simulink model "bolid_sim_2"  (R2026b)
settings: Solver=ode23t  StopTime=180
model workspace (MAT data in the model file):
  sample_time = 0.001
libraries: fl_lib x19, nesl_utility x14, ee_lib x6, slpidlib x2, simulink x1, sdl_lib x1
settings Model: Creator=LH213  LastModifiedBy=stycz
settings RTWCC: GPUComputeCapability=5.0
settings SimscapeCC: SimscapeUseEnergyAccounting=off

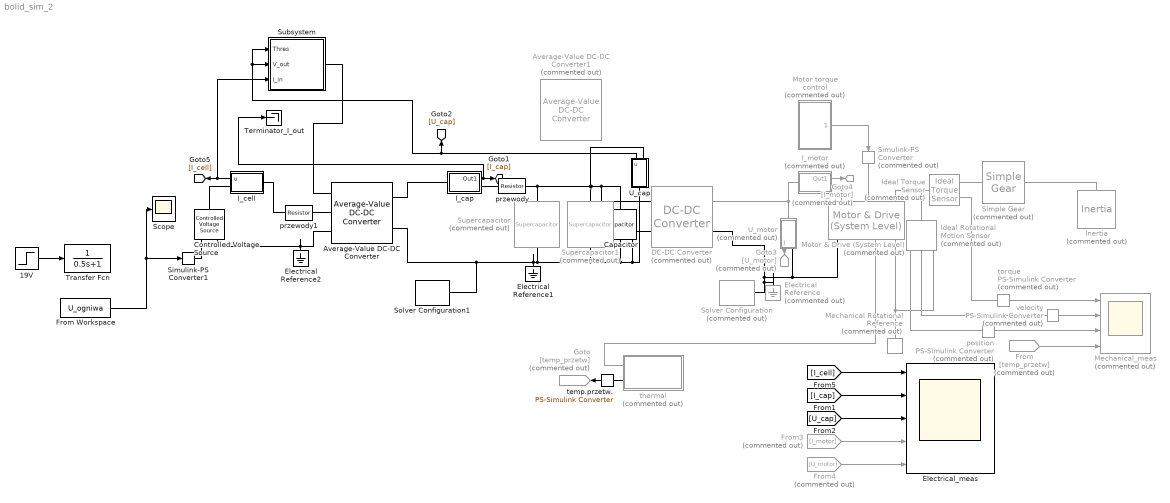
== system bolid_sim_2 ==
  19V : Step  Time=0  FinalValue=19  SampleTime=0
  Average-Value DC-DC Converter : ee_lib/Semiconductors & Converters/Converters/Average-Value DC-DC Converter  implementation_option=ee.enum.converters.implementation.behavioral  converter_type=ee.enum.converters.dcdctype.buckboost  control_option=ee.enum.converters.controlinput.dutycycle  efficiency_option=ee.enum.converters.efficiency.constant  efficiency_fixed=85  i_vec=[0, 2, 5] A  efficiency_vec=[90, 95, 98]  Lf=1e-6 H  Rl=0 Ohm  Cf=1e-7 F  Rc=1e-6 Ohm  iL_specify=off  iL_priority=High  iL=0 A  iL_nominal_specify=off  iL_nominal_value=1  iL_nominal_unit=A  vc_specify=off  vc_priority=High  vc=0 V  vc_nominal_specify=off  vc_nominal_value=1  vc_nominal_unit=V
  Average-Value DC-DC Converter1 : ee_lib/Semiconductors & Converters/Converters/Average-Value DC-DC Converter  Commented=on  implementation_option=ee.enum.converters.implementation.averageValue  converter_type=ee.enum.converters.dcdctype.buckboost  control_option=ee.enum.converters.controlinput.dutycycle  efficiency_option=ee.enum.converters.efficiency.constant  efficiency_fixed=100  i_vec=[0, 2, 5] A  efficiency_vec=[90, 95, 98]  Lf=1e-6 H  Rl=0 Ohm  Cf=1e-7 F  Rc=1e-6 Ohm  iL_specify=off  iL_priority=High  iL=0 A  iL_nominal_specify=off  iL_nominal_value=1  iL_nominal_unit=A  vc_specify=off  vc_priority=High  vc=0 V  vc_nominal_specify=off  vc_nominal_value=1  vc_nominal_unit=V
  Capacitor : fl_lib/Electrical/Electrical Elements/Capacitor  c=0.5 F  r=0.022 Ohm  g=0 1/Ohm  i_specify=off  i_priority=None  i=0 A  i_nominal_specify=off  i_nominal_value=1  i_nominal_unit=A  v_specify=off  v_priority=None  v=0 V  v_nominal_specify=off  v_nominal_value=1  v_nominal_unit=V  vc_specify=on  vc_priority=High  vc=0 V  vc_nominal_specify=off  vc_nominal_value=1  vc_nominal_unit=V
  Controlled Voltage Source : fl_lib/Electrical/Electrical Sources/Controlled Voltage Source
  DC-DC Converter : ee_lib/Semiconductors & Converters/Converters/DC-DC Converter  Commented=on  Vref_option=ee.enum.converters.voltageref.internal  v_ref=10 V  P_rated=10 W  droop_enabled=true  droop_param=ee.enum.converters.droop.value  droop=0.1 V/A  droop_percent=2  Vref_droop=10 V  reversible=ee.enum.converters.directionality.unidirectional  G_diode=1e-8 1/Ohm  P_fixed=1 W  losses_option=ee.enum.converters.lossesOption.proportionalToSquaredCurrent  eff_rated=80  tableOption=ee.enum.converters.lossTableOptionThermal.currentTemp  i_eff_vec=[-2, -1, 1, 2] A  v_eff_vec=[15, 30, 45] V  eff_vec=[66, 76, 80, 74]  eff_2D_table=[66, 66, 66; 76, 76, 76; 80, 80, 80; 74, 74, 74]  model_dynamics=ee.enum.converters.dynamics.no  tau=0.02 s  v_ini=10 V  v1_min=1 V  R1=1000 Ohm  R2=1000 Ohm  T_eff_vec=[280, 300, 320] K  eff_3D_table=repmat([66; 76; 80; 74], 1, 3, 3)  thermal_mass=100 J/K  initial_temperature=298.15 K
  Electrical Reference : fl_lib/Electrical/Electrical Elements/Electrical Reference  Commented=on
  Electrical Reference1 : fl_lib/Electrical/Electrical Elements/Electrical Reference
  Electrical Reference2 : fl_lib/Electrical/Electrical Elements/Electrical Reference
  Electrical_meas : Scope  NumInputPorts=5
      settings: ActiveDisplayYMinimum=-6.7608311518799447  ActiveDisplayYMaximum=14.501835831634169
  From : From  Commented=on  GotoTag=temp_przetw
  From Workspace : FromWorkspace  VariableName=U_ogniwa
  From3 : From  Commented=on  GotoTag=I_motor
  From4 : From  Commented=on  GotoTag=U_motor
  Goto : Goto  Commented=on  GotoTag=temp_przetw
  Goto3 : Goto  Commented=on  GotoTag=U_motor
  Goto4 : Goto  Commented=on  GotoTag=I_motor
  I_cap : Subsystem
  I_cell : Subsystem
      settings: PortSchema="{\"entries\":[{\"content\":{\"sides\":[{\"content\":{\"connectorIds\":[\"Out1\",\"LConn1\"]},\"type\":\"ConnectorPlacement.EquallySpacedRectSide\",\"uuid\":\"769e0237-35ee-429e-8d15-01efa26456ad\"},{\"content\":{\"connectorIds\":[\"RConn1\"],\"side\":\"RIGHT\"},\"type\":\"ConnectorPlacement.EquallySpacedRectSide\",\"uuid\":\"f378939b-7465-400e-9a94-5995790dc0ac\"},{\"content\":{\"side\":\"TOP\"},\"type\":\"ConnectorPlacement.EquallySpacedRectSide\",\"uuid\":\"cbf7c360-3cb9-4610-b4dc-eb02055b4ae7\"}]},\"type\":\"ConnectorPlacement.EquallySpacedConnector\",\"uuid\":\"054beea7-831e-4463-a8af-6e4ec75c9837\"}],\"packageUris\":[\"http://schema.mathworks.com/mf0/Connector/R2020b\"],\"version\":\"1.0\"}"
  I_motor : Subsystem  Commented=on
  Ideal Rotational Motion Sensor : fl_lib/Mechanical/Mechanical Sensors/Ideal Rotational Motion Sensor  Commented=on  reference=foundation.enum.MeasurementReference.difference  acceleration_port=false  velocity_port=true  position_port=true  wrap_angle=false  offset=0 rad
  Ideal Torque Sensor : fl_lib/Mechanical/Mechanical Sensors/Ideal Torque Sensor  Commented=on
  Inertia : fl_lib/Mechanical/Rotational Elements/Inertia  Commented=on  inertia=0.3 kg*m^2  num_ports=foundation.enum.numPorts2.one  w_specify=off  w_priority=High  w=0 rad/s  w_nominal_specify=off  w_nominal_value=1  w_nominal_unit=rad/s  t_specify=off  t_priority=None  t=0 N*m  t_nominal_specify=off  t_nominal_value=1  t_nominal_unit=N*m
  Mechanical Rotational Reference : fl_lib/Mechanical/Rotational Elements/Mechanical Rotational Reference  Commented=on
  Mechanical_meas : Scope  Commented=on  NumInputPorts=4
      settings: ActiveDisplayYMinimum=-1  ActiveDisplayYMaximum=1
  Motor & Drive (System Level) : ee_lib/Electromechanical/Motor & Drive (System Level)  Commented=on  torque_speed_param=ee.enum.electromech.envelope.tabulated  overtorque_param=ee.enum.electromech.overtorque.no  T_t=[.09, .08, .07, 0] N*m  T_t_intermittent=[.36, .32, .28, 0] N*m  T_t_2D=[.09, .09, .09; .08, .08, .08; .07, .07, .07; 0, 0, 0] N*m  T_t_intermittent_2D=[.36, .36, .36; .32, .32, .32; .28, .28, .28; 0, 0, 0] N*m  w_t=[0, 3750, 7500, 8000] rpm  vdc_t=[6, 12, 24] V  torque_max=0.1 N*m  power_max=30 W  torque_max_intermittent=0.4 N*m  power_max_intermittent=120 W  time_overtorque=30 s  time_recover=60 s  Tc=0.02 s  EnableSwitch=false  losses_param=1  eff=100  w_eff=3750 rpm  T_eff=0.08 N*m  Piron=0 W  Pbase=0 W  w_eff_vec=[-8000, -4000, 0, 4000, 8000] rpm  T_eff_vec=[0, .03, .06, .09] N*m  v_eff_vec=[100, 250, 400] V  losses_mat=[1.49, 1.67, 2.21, 3.1; .42, .69, 1.14, 2.03; .06, .24, .78, 1.68; .42, .69, 1.14, 2.03; 1.49, 1.67, 2.21, 3.1] W  efficiency_mat=[95, 95, 95, 95; 95, 95, 95, 95; 95, 95, 95, 95; 95, 95, 95, 95; 95, 95, 95, 95]  losses_mat_3D=ones(5, 4, 3) W  efficiency_mat_3D=95 * ones(5, 4, 3)  Res=0 Ohm  J=5e-6 kg*m^2  lam=1e-5 N*m*s/rad  speed0=0 rpm  faulted_specify=off  faulted_priority=None  faulted=0  faulted_nominal_specify=off  faulted_nominal_value=1  faulted_nominal_unit=1  isSwitchedOff_specify=off  isSwitchedOff_priority=None  isSwitchedOff=0  isSwitchedOff_nominal_specify=off  isSwitchedOff_nominal_value=1  isSwitchedOff_nominal_unit=1  torqueLimitContinuous_specify=off  torqueLimitContinuous_priority=None  torqueLimitContinuous=0 N*m  torqueLimitContinuous_nominal_specify=off  torqueLimitContinuous_nominal_value=1  torqueLimitContinuous_nominal_unit=N*m  TabulateLossesForMultipleTemperatures=false  alpha=3.93e-3 1/K  Tmeas=25 degC  TmeasVec=[25, 75, 125] degC  Tmeas2=125 degC  losses_mat_T2=[1.49, 1.74, 2.49, 3.74; .42, .67, 1.42, 2.67; .06, .31, 1.06, 2.31; .42, .67, 1.42, 2.67; 1.49, 1.74, 2.49, 3.74] W  efficiency_mat_T2=[95, 95, 95, 95; 95, 95, 95, 95; 95, 95, 95, 95; 95, 95, 95, 95; 95, 95, 95, 95]  losses_mat_3D_T2=ones(5, 4, 3) W  efficiency_mat_3D_T2=95 * ones(5, 4, 3)  lossesMatMultipleTemperatures=ones(5, 4, 3) W  efficiencyMatMultipleTemperatures=95 * ones(5, 4, 3)  lossesMat4DMultipleTemperatures=ones(5, 4, 3, 3) W  efficiencyMat4DMultipleTemperatures=95 * ones(5, 4, 3, 3)  thermal_mass=100 J/K  initial_temperature=25 degC
  Motor torque control : Subsystem  Commented=on
  Scope : Scope
      settings: ActiveDisplayYMinimum=17.592708049714869  ActiveDisplayYMaximum=32.673570062605506  DataLoggingVariableName=ScopeData2
  Simple Gear : sdl_lib/Gears/Simple Gear  Commented=on  ratio=15  rotation_direction=sdl.enum.shaftOutputDirection.opposite  friction_model=sdl.enum.gear_efficiencies_load.off  T_noload=0.1 N*m  T_nom=5 N*m  efficiency_nom=0.8  efficiency=0.8  temperature_TLU=[280, 300, 320] K  load_TLU=[1, 5, 10] N*m  efficiency_TLU=[.95, .9, .85]  efficiency_TLU2=[.85, .8, .75; .95, .9, .85; .85, .8, .7]  w_thr=0.01 rad/s  pwr_thr=0.001 W  enable_backlash=false  hardstop_model=simscape.enum.hardstop.smooth  backlash_distance=1e-3 mm  r_base=0.1 m  transition=1e-4 mm  backlash_stiffness=1e6 N/m  backlash_damping=1e3 N*s/m  coeff_rest=0.7  v_tol=0.001 m/s  f_tol=0.001 N  tau=0.1 s  mu_visc=[0, 0] N*m*s/rad  thermal_mass=50 J/K  temperature_specify=off  temperature_priority=High  temperature=300 K  temperature_nominal_specify=off  temperature_nominal_value=1  temperature_nominal_unit=K  x_backlash_specify=off  x_backlash_priority=None  x_backlash=0 mm  x_backlash_nominal_specify=off  x_backlash_nominal_value=1  x_backlash_nominal_unit=mm  f_hardstop_specify=off  f_hardstop_priority=None  f_hardstop=0 N  f_hardstop_nominal_specify=off  f_hardstop_nominal_value=1  f_hardstop_nominal_unit=N  v_backlash_specify=off  v_backlash_priority=None  v_backlash=0 m/s  v_backlash_nominal_specify=off  v_backlash_nominal_value=1  v_backlash_nominal_unit=m/s
  Simulink-PS Converter : nesl_utility/Simulink-PS Converter  Commented=on  PhysicalDomain=network_engine_domain  SubClassName=ps_input  LeftPortType=input  RightPortType=output  PseudoPeriodic=off  Frequencies=[]  NoiseDistribution=none  NoiseParameters=[]  Unit=1  AffineConversion=off  FilteringAndDerivatives=provide  SimscapeFilterOrder=1  InputFilterTimeConstant=0.001  UdotUserProvided=0
  Simulink-PS Converter1 : nesl_utility/Simulink-PS Converter  PhysicalDomain=network_engine_domain  SubClassName=ps_input  LeftPortType=input  RightPortType=output  PseudoPeriodic=off  Frequencies=[]  NoiseDistribution=none  NoiseParameters=[]  Unit=1  AffineConversion=off  FilteringAndDerivatives=provide  SimscapeFilterOrder=1  InputFilterTimeConstant=0.001  UdotUserProvided=0
  Solver Configuration : nesl_utility/Solver Configuration  Commented=on  PhysicalDomain=network_engine_domain  SubClassName=solver  LeftPortType=input  RightPortType=generic  Tones=[]  Harmonics=[]  SimulateNoise=off  Profile=off  UseLocalSampling=off  EnableSwitchedLinearOptims=on  FrequencyDomain=off  UseCCode=off  RelTol=0.001  AbsTol=0.001  MinStep=1e-09  ToWorkspace=off  RevertToSquareIcSolve=off  NumHomotopyIterations=100  PhasorMode=off  PhasorModeNumHarmonics=1  ConsistencySolver=NEWTON_XTOL_AFTER_FTOL  CanonicalOrdering=UNORDERED  OptimizeIntermediates=UNOPTIMIZED  MulticoreSolverChoice=BACKWARD_EULER  IndexReductionMethod=DerivativeReplacement  DoDC=off  ResidualTolerance=1e-09  ConsistencyTolSource=GLOBAL  ConsistencyAbsTol=0.001  ConsistencyRelTol=0.001  ConsistencyTolFactor=0.001  UseLocalSolver=off  LocalSolverChoice=NE_BACKWARD_EULER_ADVANCER  ResolveIndetEquations=on  FunctionEvalNumThread=1  LocalSolverSampleTime=0.001  DoFixedCost=off  MaxNonlinIter=3  MaxModeIter=2  ComputeImpulses=off  ImpulseIterations=2  LinearAlgebra=auto  LinearAlgebraNumThread=0  EquationFormulation=NE_TIME_EF  DelaysMemoryBudget=1024  AutomaticFiltering=on  FilteringTimeConstant=0.001  PartitionStorageMethod=AS_NEEDED  PartitionMemoryBudget=1024  PartitionMethod=BALANCED  MultibodyUseLocalSolver=off  MultibodyLocalSolverChoice=ODE1  MultibodyLocalSolverSampleTime=0.001
  Solver Configuration1 : nesl_utility/Solver Configuration  PhysicalDomain=network_engine_domain  SubClassName=solver  LeftPortType=input  RightPortType=generic  Tones=[]  Harmonics=[]  SimulateNoise=off  Profile=off  UseLocalSampling=off  EnableSwitchedLinearOptims=on  FrequencyDomain=off  UseCCode=off  RelTol=0.001  AbsTol=0.001  MinStep=1e-09  ToWorkspace=off  RevertToSquareIcSolve=off  NumHomotopyIterations=100  PhasorMode=off  PhasorModeNumHarmonics=1  ConsistencySolver=NEWTON_XTOL_AFTER_FTOL  CanonicalOrdering=UNORDERED  OptimizeIntermediates=UNOPTIMIZED  MulticoreSolverChoice=BACKWARD_EULER  IndexReductionMethod=DerivativeReplacement  DoDC=off  ResidualTolerance=1e-09  ConsistencyTolSource=GLOBAL  ConsistencyAbsTol=0.001  ConsistencyRelTol=0.001  ConsistencyTolFactor=0.001  UseLocalSolver=off  LocalSolverChoice=NE_BACKWARD_EULER_ADVANCER  ResolveIndetEquations=on  FunctionEvalNumThread=1  LocalSolverSampleTime=0.001  DoFixedCost=off  MaxNonlinIter=3  MaxModeIter=2  ComputeImpulses=off  ImpulseIterations=2  LinearAlgebra=auto  LinearAlgebraNumThread=0  EquationFormulation=NE_TIME_EF  DelaysMemoryBudget=1024  AutomaticFiltering=on  FilteringTimeConstant=0.001  PartitionStorageMethod=AS_NEEDED  PartitionMemoryBudget=1024  PartitionMethod=BALANCED  MultibodyUseLocalSolver=off  MultibodyLocalSolverChoice=ODE1  MultibodyLocalSolverSampleTime=0.001
  Subsystem : Subsystem
  Supercapacitor : ee_lib/Passive/Supercapacitor  Commented=on  R=[0.022, 0.022, 0.022] Ohm  C=[10.8, 10.8, 10.8] F  Kv=0.95 F/V  R_discharge=inf Ohm  N_series=1  N_parallel=1  i_specify=off  i_priority=None  i=0 A  i_nominal_specify=off  i_nominal_value=1  i_nominal_unit=A  v_specify=off  v_priority=None  v=0 V  v_nominal_specify=off  v_nominal_value=1  v_nominal_unit=V  vc1_specify=off  vc1_priority=High  vc1=0 V  vc1_nominal_specify=off  vc1_nominal_value=1  vc1_nominal_unit=V  vc2_specify=off  vc2_priority=High  vc2=0 V  vc2_nominal_specify=off  vc2_nominal_value=1  vc2_nominal_unit=V  vc3_specify=off  vc3_priority=High  vc3=0 V  vc3_nominal_specify=off  vc3_nominal_value=1  vc3_nominal_unit=V
  Supercapacitor1 : ee_lib/Passive/Supercapacitor  Commented=on  R=[0.022, 0.022, 0.022] Ohm  C=[10.8, 10.8, 10.8] F  Kv=0.95 F/V  R_discharge=inf Ohm  N_series=1  N_parallel=1  i_specify=off  i_priority=None  i=0 A  i_nominal_specify=off  i_nominal_value=1  i_nominal_unit=A  v_specify=off  v_priority=None  v=0 V  v_nominal_specify=off  v_nominal_value=1  v_nominal_unit=V  vc1_specify=off  vc1_priority=High  vc1=0 V  vc1_nominal_specify=off  vc1_nominal_value=1  vc1_nominal_unit=V  vc2_specify=off  vc2_priority=High  vc2=0 V  vc2_nominal_specify=off  vc2_nominal_value=1  vc2_nominal_unit=V  vc3_specify=off  vc3_priority=High  vc3=0 V  vc3_nominal_specify=off  vc3_nominal_value=1  vc3_nominal_unit=V
  Terminator_I_out : Terminator
  Transfer Fcn : TransferFcn  Denominator=[0.5 1]
  U_cap : Subsystem
      settings: PortSchema="{\"entries\":[{\"content\":{\"sides\":[{\"content\":{\"connectorIds\":[\"Out1\",\"LConn1\"]},\"type\":\"ConnectorPlacement.EquallySpacedRectSide\",\"uuid\":\"8a2d679d-7687-468d-9438-d9d25873ae5d\"},{\"content\":{\"connectorIds\":[\"RConn1\"],\"side\":\"RIGHT\"},\"type\":\"ConnectorPlacement.EquallySpacedRectSide\",\"uuid\":\"fbb26148-5fe0-4773-9d0a-b32ffd75f150\"},{\"content\":{\"side\":\"TOP\"},\"type\":\"ConnectorPlacement.EquallySpacedRectSide\",\"uuid\":\"e5a432c3-78b7-420b-8c8f-73de39d42f28\"}]},\"type\":\"ConnectorPlacement.EquallySpacedConnector\",\"uuid\":\"06e2cb91-7546-4b55-b6e9-700e4ff7195a\"}],\"packageUris\":[\"http://schema.mathworks.com/mf0/Connector/R2020b\"],\"version\":\"1.0\"}"
  U_motor : Subsystem  Commented=on
  position : nesl_utility/PS-Simulink Converter  Commented=on  PhysicalDomain=network_engine_domain  SubClassName=ps_output  LeftPortType=input  RightPortType=output  PseudoPeriodic=off  Frequencies=[]  VectorFormat=inherit  Unit=rad  AffineConversion=off
  przewody : fl_lib/Electrical/Electrical Elements/Resistor  R=0.2 Ohm  i_specify=off  i_priority=None  i=0 A  i_nominal_specify=off  i_nominal_value=1  i_nominal_unit=A  v_specify=off  v_priority=None  v=0 V  v_nominal_specify=off  v_nominal_value=1  v_nominal_unit=V
  przewody1 : fl_lib/Electrical/Electrical Elements/Resistor  R=0.2 Ohm  i_specify=off  i_priority=None  i=0 A  i_nominal_specify=off  i_nominal_value=1  i_nominal_unit=A  v_specify=off  v_priority=None  v=0 V  v_nominal_specify=off  v_nominal_value=1  v_nominal_unit=V
  temp.przetw. : nesl_utility/PS-Simulink Converter  PhysicalDomain=network_engine_domain  SubClassName=ps_output  LeftPortType=input  RightPortType=output  PseudoPeriodic=off  Frequencies=[]  VectorFormat=inherit  Unit=K  AffineConversion=off
  thermal : Subsystem  Commented=on
  torque : nesl_utility/PS-Simulink Converter  Commented=on  PhysicalDomain=network_engine_domain  SubClassName=ps_output  LeftPortType=input  RightPortType=output  PseudoPeriodic=off  Frequencies=[]  VectorFormat=inherit  Unit=N*m  AffineConversion=off
  velocity : nesl_utility/PS-Simulink Converter  Commented=on  PhysicalDomain=network_engine_domain  SubClassName=ps_output  LeftPortType=input  RightPortType=output  PseudoPeriodic=off  Frequencies=[]  VectorFormat=inherit  Unit=rad/s  AffineConversion=off
  wires:
  torque/1 -> Mechanical_meas/1
  velocity/1 -> Mechanical_meas/2
  position/1 -> Mechanical_meas/3
  Motor torque control/1(torque) -> Simulink-PS Converter/1
  From/1 -> Mechanical_meas/4
  temp.przetw./1 -> Goto/1
  [I_cap] -> Electrical_meas/2
  U_motor/1(Out1) -> Goto3/1
  I_motor/1(Out1) -> Goto4/1
  [U_cap] -> Electrical_meas/3
  From3/1 -> Electrical_meas/4
  From4/1 -> Electrical_meas/5
  U_cap/1(u) -> Subsystem/1(Thres), Subsystem/2(V_out), [U_cap]
  I_cell/1(u) -> Subsystem/3(I_in), [I_cell]
  [I_cell] -> Electrical_meas/1
  I_cap/1(Out1) -> Terminator_I_out/1, [I_cap]
  19V/1 -> Transfer Fcn/1
  From Workspace/1 -> Scope/1, Simulink-PS Converter1/1
  connections:
  Simple Gear/RConn1 -- Inertia/LConn1
  Mechanical Rotational Reference/LConn1 -- Ideal Rotational Motion Sensor/RConn1 -- Motor & Drive (System Level)/RConn4
  Motor & Drive (System Level)/LConn1 -- I_motor/RConn1
  Solver Configuration/RConn1 -- Electrical Reference/LConn1 -- DC-DC Converter/RConn2 -- U_motor/RConn1 -- Motor & Drive (System Level)/RConn1
  Simulink-PS Converter/RConn1 -- Motor & Drive (System Level)/LConn2
  Ideal Torque Sensor/RConn1 -- Simple Gear/LConn1
  Ideal Torque Sensor/LConn1 -- Ideal Rotational Motion Sensor/LConn1 -- Motor & Drive (System Level)/LConn3
  Ideal Rotational Motion Sensor/RConn3 -- position/LConn1
  Ideal Torque Sensor/RConn2 -- torque/LConn1
  Ideal Rotational Motion Sensor/RConn2 -- velocity/LConn1
  U_cap/RConn1 -- DC-DC Converter/LConn2 -- Capacitor/RConn1 -- Average-Value DC-DC Converter/RConn2 -- Solver Configuration1/RConn1 -- Electrical Reference1/LConn1 -- Supercapacitor/RConn1 -- Supercapacitor1/RConn1
  Average-Value DC-DC Converter/LConn3 -- Controlled Voltage Source/RConn2 -- Electrical Reference2/LConn1
  Motor & Drive (System Level)/RConn3 -- thermal/LConn1
  temp.przetw./LConn1 -- thermal/LConn2
  Average-Value DC-DC Converter/RConn1 -- I_cap/LConn1
  Controlled Voltage Source/LConn1 -- I_cell/LConn1
  Average-Value DC-DC Converter/LConn1 -- Subsystem/RConn1
  U_motor/LConn1 -- I_motor/LConn1 -- DC-DC Converter/RConn1
  I_cap/RConn1 -- przewody/LConn1
  przewody/RConn1 -- Capacitor/LConn1 -- DC-DC Converter/LConn1 -- Supercapacitor1/LConn1 -- U_cap/LConn1 -- Supercapacitor/LConn1
  przewody1/RConn1 -- Average-Value DC-DC Converter/LConn2
  przewody1/LConn1 -- I_cell/RConn1
  Controlled Voltage Source/RConn1 -- Simulink-PS Converter1/RConn1

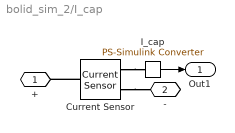
== system bolid_sim_2/I_cap ==
  Current Sensor : fl_lib/Electrical/Electrical Sensors/Current Sensor
  I_cap : nesl_utility/PS-Simulink Converter  PhysicalDomain=network_engine_domain  SubClassName=ps_output  LeftPortType=input  RightPortType=output  PseudoPeriodic=off  Frequencies=[]  VectorFormat=inherit  Unit=A  AffineConversion=off
  + : PMIOPort  Side=Left
  - : PMIOPort  Port=2  Side=Right
  Out1 : Outport
  wires:
  I_cap/1 -> Out1/1
  connections:
  Current Sensor/RConn1 -- I_cap/LConn1
  Current Sensor/RConn2 -- -/RConn1
  Current Sensor/LConn1 -- +/RConn1

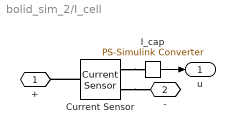
== system bolid_sim_2/I_cell ==
  Current Sensor : fl_lib/Electrical/Electrical Sensors/Current Sensor
  I_cap : nesl_utility/PS-Simulink Converter  PhysicalDomain=network_engine_domain  SubClassName=ps_output  LeftPortType=input  RightPortType=output  PseudoPeriodic=off  Frequencies=[]  VectorFormat=inherit  Unit=A  AffineConversion=off
  + : PMIOPort  Side=Left
  - : PMIOPort  Port=2  Side=Right
  u : Outport
  wires:
  I_cap/1 -> u/1
  connections:
  Current Sensor/RConn1 -- I_cap/LConn1
  Current Sensor/RConn2 -- -/RConn1
  Current Sensor/LConn1 -- +/RConn1

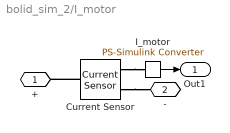
== system bolid_sim_2/I_motor ==
  Current Sensor : fl_lib/Electrical/Electrical Sensors/Current Sensor
  I_motor : nesl_utility/PS-Simulink Converter  PhysicalDomain=network_engine_domain  SubClassName=ps_output  LeftPortType=input  RightPortType=output  PseudoPeriodic=off  Frequencies=[]  VectorFormat=inherit  Unit=A  AffineConversion=off
  + : PMIOPort  Side=Left
  - : PMIOPort  Port=2  Side=Right
  Out1 : Outport
  wires:
  I_motor/1 -> Out1/1
  connections:
  Current Sensor/RConn1 -- I_motor/LConn1
  Current Sensor/RConn2 -- -/RConn1
  Current Sensor/LConn1 -- +/RConn1

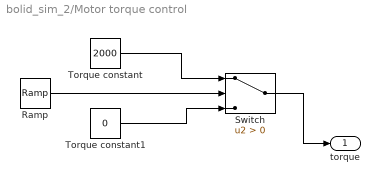
== system bolid_sim_2/Motor torque control ==
  Ramp : simulink/Sources/Ramp  slope=1  start=1  InitialOutput=0
  Switch : Switch  Criteria=u2 > Threshold  SaturateOnIntegerOverflow=off  InputSameDT=off
  Torque constant : Constant  Value=2000
  Torque constant1 : Constant  Value=0
  torque : Outport
  wires:
  Torque constant/1 -> Switch/1
  Torque constant1/1 -> Switch/3
  Ramp/1 -> Switch/2
  Switch/1 -> torque/1

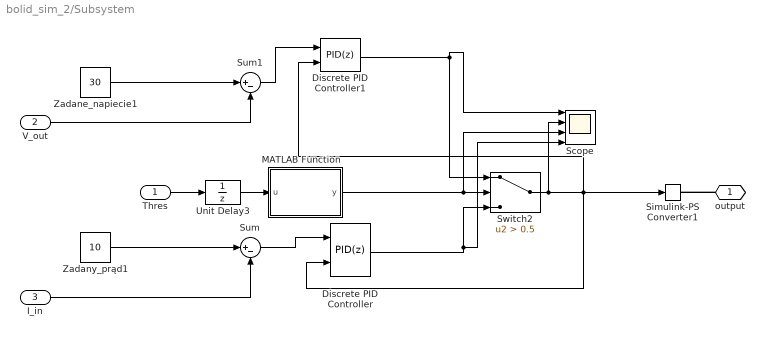
== system bolid_sim_2/Subsystem ==
  Thres : Inport
  V_out : Inport  Port=2
  I_in : Inport  Port=3
  Discrete PID Controller : slpidlib/PID Controller  Controller=PID  Form=Parallel  TimeDomain=Discrete-time  UseExternalTs=off  SampleTime=1e-3  IntegratorMethod=Forward Euler  FilterMethod=Forward Euler  ControllerParametersSource=internal  P=0.000  I=0.5  UseKiTs=off  D=0  UseExternalDerivativeSource=off  N=100  UseFilter=on  TunerSelectOption=Frequency Response Based  InitialConditionSource=internal  InitialConditionForIntegrator=0  InitialConditionForFilter=0.1  DifferentiatorICPrevScaledInput=0  ExternalReset=none  TrackingMode=on  Kt=100  LimitOutput=on  SatLimitsSource=internal  UpperSaturationLimit=0.95  LowerSaturationLimit=0  LinearizeAsGain=on  AntiWindupMode=clamping  Kb=1  LimitIntegrator=off  UpperIntegratorSaturationLimit=inf  LowerIntegratorSaturationLimit=-inf  POutMin=[]  POutMax=[]  IOutMin=[]  IOutMax=[]  DOutMin=[]  DOutMax=[]  NOutMin=[]  NOutMax=[]  SumOutMin=[]  SumOutMax=[]  SaturationOutMin=[]  SaturationOutMax=[]  PParamMin=[]  PParamMax=[]  IParamMin=[]  IParamMax=[]  DParamMin=[]  DParamMax=[]  NParamMin=[]  NParamMax=[]  KbParamMin=[]  KbParamMax=[]  KtParamMin=[]  KtParamMax=[]  KbOutMin=[]  KbOutMax=[]  KtOutMin=[]  KtOutMax=[]  IntegratorOutMin=[]  IntegratorOutMax=[]  FilterOutMin=[]  FilterOutMax=[]  SumI1OutMin=[]  SumI1OutMax=[]  SumI2OutMin=[]  SumI2OutMax=[]  SumI3OutMin=[]  SumI3OutMax=[]  SumI4OutMin=[]  SumI4OutMax=[]  SumDOutMin=[]  SumDOutMax=[]  DifferentiatorOutMin=[]  DifferentiatorOutMax=[]  FilterDiffOutCoefMin=[]  FilterDiffOutCoefMax=[]  ReciprocalOutMin=[]  ReciprocalOutMax=[]  SumDenOutMin=[]  SumDenOutMax=[]  SumNumOutMin=[]  SumNumOutMax=[]  DivideOutMin=[]  DivideOutMax=[]  UdiffTsProdOutMin=[]  UdiffTsProdOutMax=[]  NTsProdOutMin=[]  NTsProdOutMax=[]  UintegralTsProdOutMin=[]  UintegralTsProdOutMax=[]  UngainTsProdOutMin=[]  UngainTsProdOutMax=[]  ClampingZeroOutDataTypeStr=Inherit: Inherit via back propagation  ClampingZeroOutMin=[]  ClampingZeroOutMax=[]  FilterDenConstantOutDataTypeStr=Inherit: Inherit via back propagation  FilterDenConstantOutMin=[]  FilterDenConstantOutMax=[]  PCopyOutDataTypeStr=Inherit: Inherit via back propagation  PCopyOutMin=[]  PCopyOutMax=[]  NCopyOutDataTypeStr=Inherit: Inherit via back propagation  NCopyOutMin=[]  NCopyOutMax=[]  IntegratorContinuousStateAttributes=''  IntegratorStateMustResolveToSignalObject=off  IntegratorRTWStateStorageClass=Auto  FilterContinuousStateAttributes=''  FilterStateMustResolveToSignalObject=off  FilterRTWStateStorageClass=Auto  ParallelPVariant=InternalParameters  IdealPVariant=Disabled  IVariant=InternalParameters  DVariant=InternalParameters  IntegratorVariant=Discrete  SatVariant=Enabled  AWVariant=DiscClampingParallel  PCopyVariant=Disabled  TRVariant=Enabled  FdbkBlocksVariant=Forward  IdealPFdbkVariant=Disabled  SatFdbkVariant=Disabled  DerivativeFilterVariant=ForwardEulerFilter  NVariant=InternalParameters  NCopyVariant=Disabled  FilterICVariant=InternalICsFilter  IntegratorICVariant=InternalICs  ExternalResetVariant=Disabled  TRSumVariant=TrackingMode  SumFdbkVariant=Disabled  SumVariant=Sum_PID  TsampFilterVariant=InternalTs  TsampNgainVariant=Passthrough  TsampIntegralVariant=Disabled_SignalSpec  ExternalSaturationOutDataTypeStr=Inherit: Same as second input  DerivativeSourceVariant=ErrorSignal  PreIntVariant=InternalPreInt
      settings: LibrarySourceBlock=simulink/Discrete/Discrete PID Controller
  Discrete PID Controller1 : slpidlib/PID Controller  Controller=PID  Form=Parallel  TimeDomain=Discrete-time  UseExternalTs=off  SampleTime=1e-3  IntegratorMethod=Forward Euler  FilterMethod=Forward Euler  ControllerParametersSource=internal  P=0.02  I=0.8  UseKiTs=off  D=0  UseExternalDerivativeSource=off  N=100  UseFilter=on  TunerSelectOption=Frequency Response Based  InitialConditionSource=internal  InitialConditionForIntegrator=0.1  InitialConditionForFilter=0.1  DifferentiatorICPrevScaledInput=0  ExternalReset=none  TrackingMode=on  Kt=100  LimitOutput=on  SatLimitsSource=internal  UpperSaturationLimit=0.95  LowerSaturationLimit=0  LinearizeAsGain=off  AntiWindupMode=clamping  Kb=1  LimitIntegrator=off  UpperIntegratorSaturationLimit=inf  LowerIntegratorSaturationLimit=-inf  POutMin=[]  POutMax=[]  IOutMin=[]  IOutMax=[]  DOutMin=[]  DOutMax=[]  NOutMin=[]  NOutMax=[]  SumOutMin=[]  SumOutMax=[]  SaturationOutMin=[]  SaturationOutMax=[]  PParamMin=[]  PParamMax=[]  IParamMin=[]  IParamMax=[]  DParamMin=[]  DParamMax=[]  NParamMin=[]  NParamMax=[]  KbParamMin=[]  KbParamMax=[]  KtParamMin=[]  KtParamMax=[]  KbOutMin=[]  KbOutMax=[]  KtOutMin=[]  KtOutMax=[]  IntegratorOutMin=[]  IntegratorOutMax=[]  FilterOutMin=[]  FilterOutMax=[]  SumI1OutMin=[]  SumI1OutMax=[]  SumI2OutMin=[]  SumI2OutMax=[]  SumI3OutMin=[]  SumI3OutMax=[]  SumI4OutMin=[]  SumI4OutMax=[]  SumDOutMin=[]  SumDOutMax=[]  DifferentiatorOutMin=[]  DifferentiatorOutMax=[]  FilterDiffOutCoefMin=[]  FilterDiffOutCoefMax=[]  ReciprocalOutMin=[]  ReciprocalOutMax=[]  SumDenOutMin=[]  SumDenOutMax=[]  SumNumOutMin=[]  SumNumOutMax=[]  DivideOutMin=[]  DivideOutMax=[]  UdiffTsProdOutMin=[]  UdiffTsProdOutMax=[]  NTsProdOutMin=[]  NTsProdOutMax=[]  UintegralTsProdOutMin=[]  UintegralTsProdOutMax=[]  UngainTsProdOutMin=[]  UngainTsProdOutMax=[]  ClampingZeroOutDataTypeStr=Inherit: Inherit via back propagation  ClampingZeroOutMin=[]  ClampingZeroOutMax=[]  FilterDenConstantOutDataTypeStr=Inherit: Inherit via back propagation  FilterDenConstantOutMin=[]  FilterDenConstantOutMax=[]  PCopyOutDataTypeStr=Inherit: Inherit via back propagation  PCopyOutMin=[]  PCopyOutMax=[]  NCopyOutDataTypeStr=Inherit: Inherit via back propagation  NCopyOutMin=[]  NCopyOutMax=[]  IntegratorContinuousStateAttributes=''  IntegratorStateMustResolveToSignalObject=off  IntegratorRTWStateStorageClass=Auto  FilterContinuousStateAttributes=''  FilterStateMustResolveToSignalObject=off  FilterRTWStateStorageClass=Auto  ParallelPVariant=InternalParameters  IdealPVariant=Disabled  IVariant=InternalParameters  DVariant=InternalParameters  IntegratorVariant=Discrete  SatVariant=Enabled  AWVariant=DiscClampingParallel  PCopyVariant=Disabled  TRVariant=Enabled  FdbkBlocksVariant=Forward  IdealPFdbkVariant=Disabled  SatFdbkVariant=Disabled  DerivativeFilterVariant=ForwardEulerFilter  NVariant=InternalParameters  NCopyVariant=Disabled  FilterICVariant=InternalICsFilter  IntegratorICVariant=InternalICs  ExternalResetVariant=Disabled  TRSumVariant=TrackingMode  SumFdbkVariant=Disabled  SumVariant=Sum_PID  TsampFilterVariant=InternalTs  TsampNgainVariant=Passthrough  TsampIntegralVariant=Disabled_SignalSpec  ExternalSaturationOutDataTypeStr=Inherit: Same as second input  DerivativeSourceVariant=ErrorSignal  PreIntVariant=InternalPreInt
      settings: LibrarySourceBlock=simulink/Discrete/Discrete PID Controller
  MATLAB Function : MATLAB Function  TreatAsAtomicUnit=on
  Scope : Scope  NumInputPorts=4
      settings: ActiveDisplayYMinimum=0.039914463799644917  ActiveDisplayYMaximum=1.0319419040032598  DataLoggingVariableName=ScopeData3
  Simulink-PS Converter1 : nesl_utility/Simulink-PS Converter  PhysicalDomain=network_engine_domain  SubClassName=ps_input  LeftPortType=input  RightPortType=output  PseudoPeriodic=off  Frequencies=[]  NoiseDistribution=none  NoiseParameters=[]  Unit=1  AffineConversion=off  FilteringAndDerivatives=provide  SimscapeFilterOrder=1  InputFilterTimeConstant=0.001  UdotUserProvided=0
  Sum : Sum  Inputs=|+-
  Sum1 : Sum  Inputs=|+-
  Switch2 : Switch  Criteria=u2 > Threshold  Threshold=0.5  SaturateOnIntegerOverflow=off  InputSameDT=off
  Unit Delay3 : UnitDelay  SampleTime=1e-3
  Zadane_napiecie1 : Constant  Value=30
  Zadany_prąd1 : Constant  Value=10
  output : PMIOPort  Side=Right
  wires:
  Zadane_napiecie1/1 -> Sum1/1
  V_out/1 -> Sum1/2
  Zadany_prąd1/1 -> Sum/1
  I_in/1 -> Sum/2
  MATLAB Function/1(y) -> Switch2/2, Scope/3
  Switch2/1 -> Discrete PID Controller1/2, Discrete PID Controller/2, Simulink-PS Converter1/1, Scope/2
  Discrete PID Controller/1 -> Scope/4, Switch2/3
  Sum/1 -> Discrete PID Controller/1
  Discrete PID Controller1/1 -> Scope/1, Switch2/1
  Sum1/1 -> Discrete PID Controller1/1
  Thres/1 -> Unit Delay3/1
  Unit Delay3/1 -> MATLAB Function/1(u)
  connections:
  output/RConn1 -- Simulink-PS Converter1/RConn1

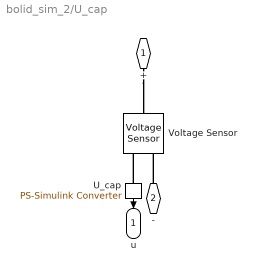
== system bolid_sim_2/U_cap ==
  U_cap : nesl_utility/PS-Simulink Converter  PhysicalDomain=network_engine_domain  SubClassName=ps_output  LeftPortType=input  RightPortType=output  PseudoPeriodic=off  Frequencies=[]  VectorFormat=inherit  Unit=V  AffineConversion=off
  Voltage Sensor : fl_lib/Electrical/Electrical Sensors/Voltage Sensor
  + : PMIOPort  Side=Left
  - : PMIOPort  Port=2  Side=Right
  u : Outport
  wires:
  U_cap/1 -> u/1
  connections:
  -/RConn1 -- Voltage Sensor/RConn2
  U_cap/LConn1 -- Voltage Sensor/RConn1
  +/RConn1 -- Voltage Sensor/LConn1

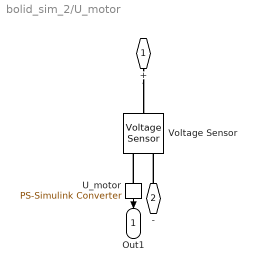
== system bolid_sim_2/U_motor ==
  U_motor : nesl_utility/PS-Simulink Converter  PhysicalDomain=network_engine_domain  SubClassName=ps_output  LeftPortType=input  RightPortType=output  PseudoPeriodic=off  Frequencies=[]  VectorFormat=inherit  Unit=V  AffineConversion=off
  Voltage Sensor : fl_lib/Electrical/Electrical Sensors/Voltage Sensor
  + : PMIOPort  Side=Left
  - : PMIOPort  Port=2  Side=Right
  Out1 : Outport
  wires:
  U_motor/1 -> Out1/1
  connections:
  -/RConn1 -- Voltage Sensor/RConn2
  U_motor/LConn1 -- Voltage Sensor/RConn1
  +/RConn1 -- Voltage Sensor/LConn1

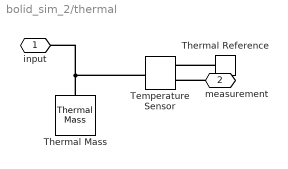
== system bolid_sim_2/thermal ==
  Temperature Sensor : fl_lib/Thermal/Thermal Sensors/Temperature Sensor  temperature_measure=foundation.enum.MeasurementReference.difference
  Thermal Mass : fl_lib/Thermal/Thermal Elements/Thermal Mass  mass_type=foundation.enum.constant_variable.constant  mass=1 kg  sp_heat=447 J/(K*kg)  mass_min=1e-6 kg  num_ports=foundation.enum.numPorts2.one  m_specify=off  m_priority=High  m=1 kg  m_nominal_specify=off  m_nominal_value=1  m_nominal_unit=kg  T_specify=off  T_priority=High  T=300 K  T_nominal_specify=off  T_nominal_value=1  T_nominal_unit=K  Q_specify=off  Q_priority=None  Q=0 W  Q_nominal_specify=off  Q_nominal_value=1  Q_nominal_unit=W
  Thermal Reference : fl_lib/Thermal/Thermal Elements/Thermal Reference
  input : PMIOPort  Side=Left
  measurement : PMIOPort  Port=2  Side=Left
  connections:
  Temperature Sensor/LConn1 -- input/RConn1 -- Thermal Mass/LConn1
  Thermal Reference/LConn1 -- Temperature Sensor/RConn1
  measurement/RConn1 -- Temperature Sensor/RConn2

== matlab function bolid_sim_2/Subsystem/MATLAB Function ==
  data: u input; y output
function y = fcn(u)
persistent state;
if isempty(state)
    state = 0; % Start w trybie prądowym (wejście F w Switch)
end

if u > 30.05
    state = 1; % Przejście na stabilizację napięcia (wejście T w Switch)
elseif u < 29.5
    state = 0; % Powrót do ładowania stałym prądem (wejście F w Switch)
end

y = state;
